simulink model "mo_hinh_dwt_wiener"  (R2026b)
settings: Solver=FixedStepDiscrete  StopTime=5.2480000000000002  FixedStep=6.2500000000000001e-05
InitFcn:
  | model = bdroot;
  | roleMatches=find_system(model,'LookUnderMasks','all','FollowLinks','off','IncludeCommented','on','Tag','WaveletDSP:source');
  | assert(numel(roleMatches)==1,'WaveletDSP:Role','Thiếu hoặc trùng định danh nội bộ: source. Không cần khôi phục tên hiển thị.');
  | source=get_param(roleMatches{1},'Handle');
  | roleMatches=find_system(model,'LookUnderMasks','all','FollowLinks','off','IncludeCommented','on','Tag','WaveletDSP:clean');
  | assert(numel(roleMatches)==1,'WaveletDSP:Role','Thiếu hoặc trùng định danh nội bộ: clean. Không cần khôi phục tên hiển thị.');
  | cleanSource=get_param(roleMatches{1},'Handle');
  | roleMatches=find_system(model,'LookUnderMasks','all','FollowLinks','off','IncludeCommented','on','Tag','WaveletDSP:sink');
  | assert(numel(roleMatches)==1,'WaveletDSP:Role','Thiếu hoặc trùng định danh nội bộ: sink. Không cần khôi phục tên hiển thị.');
  | sink=get_param(roleMatches{1},'Handle');
  | roleMatches=find_system(model,'LookUnderMasks','all','FollowLinks','off','IncludeCommented','on','Tag','WaveletDSP:filter');
  | assert(numel(roleMatches)==1,'WaveletDSP:Role','Thiếu hoặc trùng định danh nội bộ: filter. Không cần khôi phục tên hiển thị.');
  | filterBlock=get_param(roleMatches{1},'Handle');
  | roleMatches=find_system(model,'LookUnderMasks','all','FollowLinks','off','IncludeCommented','on','Tag','WaveletDSP:reference_sync');
  | assert(numel(roleMatches)==1,'WaveletDSP:Role','Thiếu hoặc trùng định danh nội bộ: reference_sync. Không cần khôi phục tên hiển thị.');
  | referenceSync=get_param(roleMatches{1},'Handle');
  | roleMatches=find_system(model,'LookUnderMasks','all','FollowLinks','off','IncludeCommented','on','Tag','WaveletDSP:noisy_sync');
  | assert(numel(roleMatches)==1,'WaveletDSP:Role','Thiếu hoặc trùng định danh nội bộ: noisy_sync. Không cần khôi phục tên hiển thị.');
  | noisySync=get_param(roleMatches{1},'Handle');
  | workspace = get_param(model,'ModelWorkspace');
  | assignin(workspace,'Export_Complete',false);
  | inputFile = get_param(source,'inputFilename');
  | inputInfo = audioinfo(inputFile);
  | assert(inputInfo.NumChannels==1,'Chỉ hỗ trợ âm thanh một kênh.');
  | useClean = strcmp(get_param(filterBlock,'Use_Clean'),'1');
  | cleanFile = get_param(cleanSource,'inputFilename');
  | if useClean && strcmp(get_param(filterBlock,'Auto_Clean'),'1')
  |     [inputFolder,inputStem] = fileparts(inputFile);
  |     recordId = regexp(inputStem,'^(speech_\d+)_','tokens','once');
  |     assert(~isempty(recordId),'Không tìm được âm thanh sạch; tắt ghép tệp tự động và chọn tệp tham chiếu trực tiếp.');
  |     cleanFile = fullfile(fileparts(fileparts(inputFolder)),'clean',[recordId{1} '.wav']);
  | end
  | frameSize = str2double(get_param(source,'SamplesPerFrame'));
  | assert(isfinite(frameSize) && frameSize>0 && mod(frameSize,128)==0,'Số mẫu mỗi khung âm thanh có nhiễu phải là bội dương của 128.');
  | if useClean
  |     cleanInfo = audioinfo(cleanFile);
  |     assert(cleanInfo.SampleRate==inputInfo.SampleRate && cleanInfo.TotalSamples==inputInfo.TotalSamples && cleanInfo.NumChannels==1,'Âm thanh sạch/noisy must match sample rate and length.');
  |     if ~strcmp(get_param(filterBlock,'Auto_Frame'),'1')
  |         assert(str2double(get_param(cleanSource,'SamplesPerFrame'))==frameSize,'Âm thanh sạch/Noisy frame sizes differ. Set them explicitly or enable Auto_Frame.');
  |     end
  | end
  | levels = [1 2 3 4 5 6 7 7];
  | powerWindow = str2double(get_param(filterBlock,'Win_Pow'));
  | smoothWindow = str2double(get_param(filterBlock,'Win_Smooth'));
  | powerLengths = max(1,round(powerWindow*inputInfo.SampleRate./2.^levels));
  | smoothLengths = max(1,round(smoothWindow*inputInfo.SampleRate./2.^levels));
  | bandDelays = floor((powerLengths-1)/2)+floor((smoothLengths-1)/2);
  | totalDelay = 29*(2^7-1)+128*ceil(max(bandDelays.*2.^levels)/128);
  | frameCount = ceil((inputInfo.TotalSamples+totalDelay)/frameSize);
  | requiredStop = (frameCount-1)*frameSize/inputInfo.SampleRate;
  | autoRun = strcmp(get_param(filterBlock,'Auto_Run'),'1');
  | if ~autoRun
  |     assert(strcmp(get_param(model,'Solver'),'FixedStepDiscrete'),'Chọn bộ giải rời rạc bước cố định hoặc bật tự tính thời gian mô phỏng.');
  |     stepValue = slResolve(get_param(model,'FixedStep'),model);
  |     stopValue = slResolve(get_param(model,'StopTime'),model);
  |     assert(isscalar(stepValue) && isfinite(stepValue) && stepValue>0 && stepValue<=1/inputInfo.SampleRate && abs((1/inputInfo.SampleRate)/stepValue-round((1/inputInfo.SampleRate)/stepValue))<1e-8,'Bước mô phỏng phải chia hết chu kỳ lấy mẫu; chỉnh bước hoặc bật tự tính thời gian.');
  |     assert(isscalar(stopValue) && isfinite(stopValue) && stopValue>=requiredStop,'Thời gian dừng quá ngắn hoặc vô hạn; đặt thời gian hữu hạn đủ dài hoặc bật tự tính thời gian.');
  | end
  | configuredOutput = get_param(sink,'outputFilename');
  | assert(~strcmp(inputFile,configuredOutput) && ~strcmp(cleanFile,configuredOutput),'Tệp đầu ra không được trùng tệp đầu vào.');
  | ... (+47 lines)
StopFcn:
  | model = bdroot;
  | workspace = get_param(model,'ModelWorkspace');
  | roleMatches=find_system(model,'LookUnderMasks','all','FollowLinks','off','IncludeCommented','on','Tag','WaveletDSP:sink');
  | assert(numel(roleMatches)==1,'WaveletDSP:Role','Thiếu hoặc trùng định danh nội bộ: sink. Không cần khôi phục tên hiển thị.');
  | sink=get_param(roleMatches{1},'Handle');
  | roleMatches=find_system(model,'LookUnderMasks','all','FollowLinks','off','IncludeCommented','on','Tag','WaveletDSP:clean');
  | assert(numel(roleMatches)==1,'WaveletDSP:Role','Thiếu hoặc trùng định danh nội bộ: clean. Không cần khôi phục tên hiển thị.');
  | cleanSource=get_param(roleMatches{1},'Handle');
  | outputFile = evalin(workspace,'Last_Output_File');
  | restoreSettings = evalin(workspace,'Run_Restore_Settings');
  | set_param(sink,'outputFilename',restoreSettings.OutputFile);
  | set_param(cleanSource,'inputFilename',restoreSettings.CleanFile,'Commented',restoreSettings.CleanCommented);
  | [outputAudio,outputRate] = audioread(outputFile);
  | delaySamples = evalin(workspace,'Total_Delay');
  | validSamples = evalin(workspace,'Valid_Samples');
  | assert(size(outputAudio,1)>=delaySamples+validSamples,'Mô phỏng dừng sớm: đầu ra chưa đủ mẫu; tệp thô được giữ lại.');
  | outputAudio = outputAudio(delaySamples+(1:validSamples),:);
  | audiowrite(outputFile,outputAudio,outputRate,'BitsPerSample',24);
  | assignin(workspace,'Export_Complete',true);
  | fprintf('Đã xuất âm thanh và giữ thiết lập. Tệp âm thanh: %s\n',outputFile);
model workspace (MAT data in the model file):
  Audio_Fs = 16000
  Export_Complete = 1
  Frame_Size = 1024
  Last_Output_File = '/home/alberttochiro/Documents/Codex/PRJ/WaveletDSP/results/denoised_output_20261108_091202_407.wav'
  Reference_Available = 1
  Run_Clean_File = '/home/alberttochiro/Documents/Codex/PRJ/WaveletDSP/data_DSP_speech/clean/speech_004.wav'
  Run_Restore_Settings : object (value not decoded)
  Total_Delay = 4579
  Valid_Samples = 79500
undefined symbols (not defined in the file or in its folder): dspblkCoreblockFVToolHelper, gcbh, Pn_1, Pn_2, Pn_3, Pn_4, Pn_5, Pn_6, Pn_7, Pn_8
libraries: dspvision x3, dspmlti4 x2, simulink x2
(part 2 of 2)

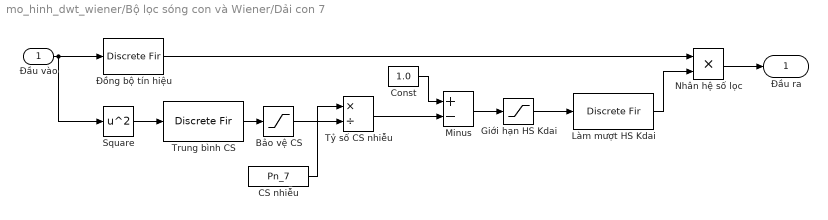
== system mo_hinh_dwt_wiener/Bộ lọc sóng con và Wiener/Dải con 7 ==
  Đầu vào : Inport
  Bảo vệ CS : Saturate  UpperLimit=inf  LowerLimit=realmin
  CS nhiễu : Constant  Value=Pn_7
  Const : Constant  Value=1.0
  Giới hạn HS Kdai : Saturate  UpperLimit=1.0  LowerLimit=Gain_Floor
  Làm mượt HS Kdai : DiscreteFir  Tag=WaveletDSP:sm_7  Coefficients=ones(1,Sample_Count)/Sample_Count  InputProcessing=Columns as channels (frame based)  mask{Sample_Count=5}
      mask prompts: Sample_Count "Số mẫu cửa sổ (tự tính từ thiết lập bộ lọc)"
      mask help: Trung bình các mẫu trong cửa sổ. Chỉnh thời gian cửa sổ tại bộ lọc; không cần nhập dãy hệ số.
      mask init:
      | validateattributes(Sample_Count,{'double'},{'scalar','integer','finite','>=',1});
  Minus : Sum  Inputs=+-
  Nhân hệ số lọc : Product
  Square : Math  Operator=square
  Trung bình CS : DiscreteFir  Tag=WaveletDSP:pow_7  Coefficients=ones(1,Sample_Count)/Sample_Count  InputProcessing=Columns as channels (frame based)  mask{Sample_Count=8}
      mask prompts: Sample_Count "Số mẫu cửa sổ (tự tính từ thiết lập bộ lọc)"
      mask help: Trung bình các mẫu trong cửa sổ. Chỉnh thời gian cửa sổ tại bộ lọc; không cần nhập dãy hệ số.
      mask init:
      | validateattributes(Sample_Count,{'double'},{'scalar','integer','finite','>=',1});
  Tỷ số CS nhiễu : Product  Inputs=*/
  Đồng bộ tín hiệu : DiscreteFir  Tag=WaveletDSP:sync_7  Coefficients=[zeros(1,Sample_Count) 1]  InputProcessing=Columns as channels (frame based)  mask{Sample_Count=5}
      mask prompts: Sample_Count "Số mẫu đồng bộ (tự tính từ cấu trúc và thiết lập bộ lọc)"
      mask help: Đồng bộ tín hiệu theo số mẫu. Giá trị được tính tự động để giữ nguyên phép lọc; không cần nhập dãy hệ số.
      mask init:
      | validateattributes(Sample_Count,{'double'},{'scalar','integer','finite','>=',0});
  Đầu ra : Outport
  wires:
  Đầu vào/1 -> Đồng bộ tín hiệu/1, Square/1
  Square/1 -> Trung bình CS/1
  Trung bình CS/1 -> Bảo vệ CS/1
  CS nhiễu/1 -> Tỷ số CS nhiễu/1
  Bảo vệ CS/1 -> Tỷ số CS nhiễu/2
  Const/1 -> Minus/1
  Tỷ số CS nhiễu/1 -> Minus/2
  Minus/1 -> Giới hạn HS Kdai/1
  Giới hạn HS Kdai/1 -> Làm mượt HS Kdai/1
  Đồng bộ tín hiệu/1 -> Nhân hệ số lọc/1
  Làm mượt HS Kdai/1 -> Nhân hệ số lọc/2
  Nhân hệ số lọc/1 -> Đầu ra/1

== system mo_hinh_dwt_wiener/Bộ lọc sóng con và Wiener/Dải con 8 ==
  Đầu vào : Inport
  Bảo vệ CS : Saturate  UpperLimit=inf  LowerLimit=realmin
  CS nhiễu : Constant  Value=Pn_8
  Const : Constant  Value=1.0
  Giới hạn HS Kdai : Saturate  UpperLimit=1.0  LowerLimit=Gain_Floor
  Làm mượt HS Kdai : DiscreteFir  Tag=WaveletDSP:sm_8  Coefficients=ones(1,Sample_Count)/Sample_Count  InputProcessing=Columns as channels (frame based)  mask{Sample_Count=5}
      mask prompts: Sample_Count "Số mẫu cửa sổ (tự tính từ thiết lập bộ lọc)"
      mask help: Trung bình các mẫu trong cửa sổ. Chỉnh thời gian cửa sổ tại bộ lọc; không cần nhập dãy hệ số.
      mask init:
      | validateattributes(Sample_Count,{'double'},{'scalar','integer','finite','>=',1});
  Minus : Sum  Inputs=+-
  Nhân hệ số lọc : Product
  Square : Math  Operator=square
  Trung bình CS : DiscreteFir  Tag=WaveletDSP:pow_8  Coefficients=ones(1,Sample_Count)/Sample_Count  InputProcessing=Columns as channels (frame based)  mask{Sample_Count=8}
      mask prompts: Sample_Count "Số mẫu cửa sổ (tự tính từ thiết lập bộ lọc)"
      mask help: Trung bình các mẫu trong cửa sổ. Chỉnh thời gian cửa sổ tại bộ lọc; không cần nhập dãy hệ số.
      mask init:
      | validateattributes(Sample_Count,{'double'},{'scalar','integer','finite','>=',1});
  Tỷ số CS nhiễu : Product  Inputs=*/
  Đồng bộ tín hiệu : DiscreteFir  Tag=WaveletDSP:sync_8  Coefficients=[zeros(1,Sample_Count) 1]  InputProcessing=Columns as channels (frame based)  mask{Sample_Count=5}
      mask prompts: Sample_Count "Số mẫu đồng bộ (tự tính từ cấu trúc và thiết lập bộ lọc)"
      mask help: Đồng bộ tín hiệu theo số mẫu. Giá trị được tính tự động để giữ nguyên phép lọc; không cần nhập dãy hệ số.
      mask init:
      | validateattributes(Sample_Count,{'double'},{'scalar','integer','finite','>=',0});
  Đầu ra : Outport
  wires:
  Đầu vào/1 -> Đồng bộ tín hiệu/1, Square/1
  Square/1 -> Trung bình CS/1
  Trung bình CS/1 -> Bảo vệ CS/1
  CS nhiễu/1 -> Tỷ số CS nhiễu/1
  Bảo vệ CS/1 -> Tỷ số CS nhiễu/2
  Const/1 -> Minus/1
  Tỷ số CS nhiễu/1 -> Minus/2
  Minus/1 -> Giới hạn HS Kdai/1
  Giới hạn HS Kdai/1 -> Làm mượt HS Kdai/1
  Đồng bộ tín hiệu/1 -> Nhân hệ số lọc/1
  Làm mượt HS Kdai/1 -> Nhân hệ số lọc/2
  Nhân hệ số lọc/1 -> Đầu ra/1

== system mo_hinh_dwt_wiener/Bộ đo chỉ số/Mẫu hợp lệ ==
  Bảo vệ số mẫu : Saturate  UpperLimit=inf  LowerLimit=realmin
  Chỉ số mẫu : Bias  Bias=(0:Frame_Size-1)'  SaturateOnIntegerOverflow=off
  Mẫu được tính : Logic  AllPortsSameDT=off  OutDataTypeStr=boolean
  Sau điểm bắt đầu : simulink/Logic and Bit Operations/Compare To Constant  relop=>=  const=Total_Delay  OutDataTypeStr=boolean
  Thời gian khung : DigitalClock  SampleTime=Frame_Size/Audio_Fs
  Trước điểm kết thúc : simulink/Logic and Bit Operations/Compare To Constant  relop=<  const=Total_Delay+Valid_Samples  OutDataTypeStr=boolean
  Tích lũy số mẫu : DiscreteFilter  Numerator=1  Denominator=[1 -1]
  Tổng theo khung số mẫu : Gain  Gain=ones(1,Frame_Size)  Multiplication=Matrix(K*u)
  Vị trí đầu khung : Gain  Gain=Audio_Fs
  Đổi kiểu mẫu hợp lệ : DataTypeConversion  OutDataTypeStr=double  SaturateOnIntegerOverflow=off  RndMeth=Floor
  Output 1 : Outport
  Output 2 : Outport  Port=2
  Output 3 : Outport  Port=3
  wires:
  Trước điểm kết thúc/1 -> Mẫu được tính/2
  Đổi kiểu mẫu hợp lệ/1 -> Output 1/1, Tổng theo khung số mẫu/1
  Tích lũy số mẫu/1 -> Output 3/1, Bảo vệ số mẫu/1
  Tổng theo khung số mẫu/1 -> Tích lũy số mẫu/1
  Mẫu được tính/1 -> Đổi kiểu mẫu hợp lệ/1
  Vị trí đầu khung/1 -> Chỉ số mẫu/1
  Chỉ số mẫu/1 -> Sau điểm bắt đầu/1, Trước điểm kết thúc/1
  Thời gian khung/1 -> Vị trí đầu khung/1
  Sau điểm bắt đầu/1 -> Mẫu được tính/1
  Bảo vệ số mẫu/1 -> Output 2/1

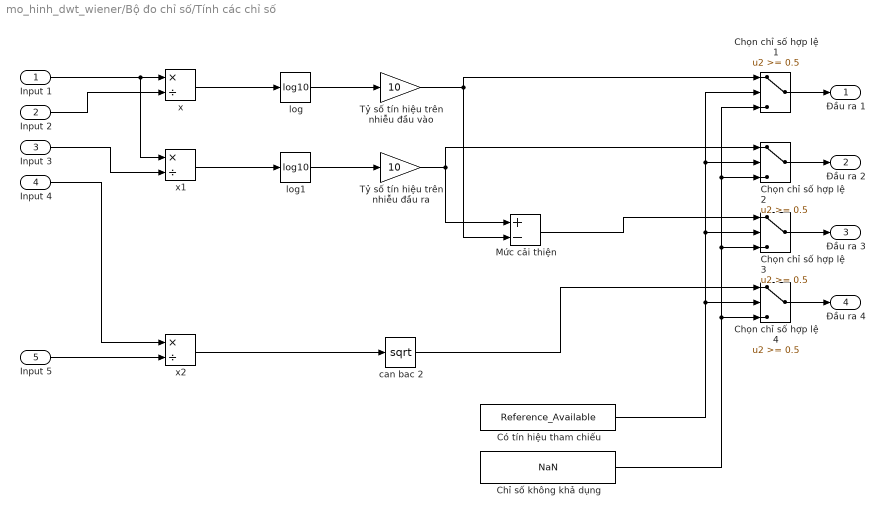
== system mo_hinh_dwt_wiener/Bộ đo chỉ số/Tính các chỉ số ==
  Input 1 : Inport
  Input 2 : Inport  Port=2
  Input 3 : Inport  Port=3
  Input 4 : Inport  Port=4
  Input 5 : Inport  Port=5
  Chỉ số không khả dụng : Constant  Value=NaN
  Chọn chỉ số hợp lệ {1..4} (4 alike) : Switch  Threshold=0.5  SaturateOnIntegerOverflow=off  InputSameDT=off
  Có tín hiệu tham chiếu : Constant  Value=Reference_Available
  Mức cải thiện : Sum  Inputs=+-
  Tỷ số tín hiệu trên nhiễu đầu ra : Gain  Gain=10
  Tỷ số tín hiệu trên nhiễu đầu vào : Gain  Gain=10
  can bac 2 : Math  Operator=sqrt
  log : Math  Operator=log10
  log1 : Math  Operator=log10
  x : Product  Inputs=*/
  x1 : Product  Inputs=*/
  x2 : Product  Inputs=*/
  Đầu ra 1 : Outport
  Đầu ra 2 : Outport  Port=2
  Đầu ra 3 : Outport  Port=3
  Đầu ra 4 : Outport  Port=4
  wires:
  x1/1 -> log1/1
  Input 3/1 -> x1/2
  Chọn chỉ số hợp lệ 4/1 -> Đầu ra 4/1
  Có tín hiệu tham chiếu/1 -> Chọn chỉ số hợp lệ 1/2, Chọn chỉ số hợp lệ 2/2, Chọn chỉ số hợp lệ 3/2, Chọn chỉ số hợp lệ 4/2
  log/1 -> Tỷ số tín hiệu trên nhiễu đầu vào/1
  Input 5/1 -> x2/2
  x/1 -> log/1
  Mức cải thiện/1 -> Chọn chỉ số hợp lệ 3/1
  Chọn chỉ số hợp lệ 2/1 -> Đầu ra 2/1
  Chọn chỉ số hợp lệ 1/1 -> Đầu ra 1/1
  Input 4/1 -> x2/1
  Chọn chỉ số hợp lệ 3/1 -> Đầu ra 3/1
  can bac 2/1 -> Chọn chỉ số hợp lệ 4/1
  Input 1/1 -> x1/1, x/1
  log1/1 -> Tỷ số tín hiệu trên nhiễu đầu ra/1
  Tỷ số tín hiệu trên nhiễu đầu ra/1 -> Mức cải thiện/1, Chọn chỉ số hợp lệ 2/1
  x2/1 -> can bac 2/1
  Tỷ số tín hiệu trên nhiễu đầu vào/1 -> Chọn chỉ số hợp lệ 1/1, Mức cải thiện/2
  Input 2/1 -> x/2
  Chỉ số không khả dụng/1 -> Chọn chỉ số hợp lệ 3/3, Chọn chỉ số hợp lệ 1/3, Chọn chỉ số hợp lệ 2/3, Chọn chỉ số hợp lệ 4/3

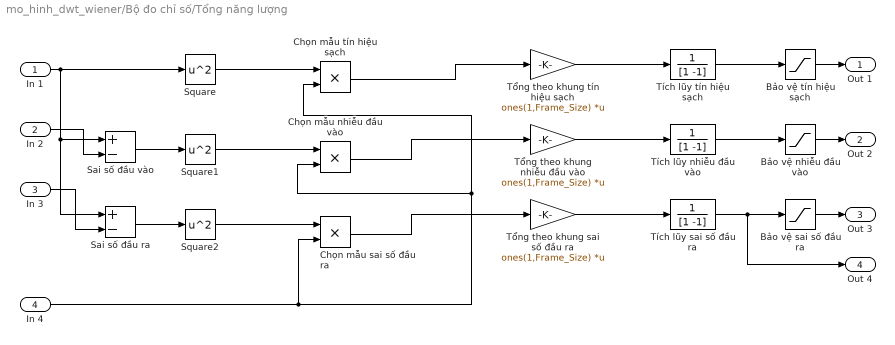
== system mo_hinh_dwt_wiener/Bộ đo chỉ số/Tổng năng lượng ==
  In 1 : Inport
  In 2 : Inport  Port=2
  In 3 : Inport  Port=3
  In 4 : Inport  Port=4
  Bảo vệ nhiễu đầu vào : Saturate  UpperLimit=inf  LowerLimit=realmin
  Bảo vệ sai số đầu ra : Saturate  UpperLimit=inf  LowerLimit=realmin
  Bảo vệ tín hiệu sạch : Saturate  UpperLimit=inf  LowerLimit=realmin
  Chọn mẫu nhiễu đầu vào : Product
  Chọn mẫu sai số đầu ra : Product
  Chọn mẫu tín hiệu sạch : Product
  Sai số đầu ra : Sum  Inputs=+-
  Sai số đầu vào : Sum  Inputs=+-
  Square : Math  Operator=square
  Square1 : Math  Operator=square
  Square2 : Math  Operator=square
  Tích lũy nhiễu đầu vào : DiscreteFilter  Numerator=1  Denominator=[1 -1]
  Tích lũy sai số đầu ra : DiscreteFilter  Numerator=1  Denominator=[1 -1]
  Tích lũy tín hiệu sạch : DiscreteFilter  Numerator=1  Denominator=[1 -1]
  Tổng theo khung nhiễu đầu vào : Gain  Gain=ones(1,Frame_Size)  Multiplication=Matrix(K*u)
  Tổng theo khung sai số đầu ra : Gain  Gain=ones(1,Frame_Size)  Multiplication=Matrix(K*u)
  Tổng theo khung tín hiệu sạch : Gain  Gain=ones(1,Frame_Size)  Multiplication=Matrix(K*u)
  Out 1 : Outport
  Out 2 : Outport  Port=2
  Out 3 : Outport  Port=3
  Out 4 : Outport  Port=4
  wires:
  Sai số đầu ra/1 -> Square2/1
  Tích lũy nhiễu đầu vào/1 -> Bảo vệ nhiễu đầu vào/1
  Chọn mẫu tín hiệu sạch/1 -> Tổng theo khung tín hiệu sạch/1
  Tích lũy tín hiệu sạch/1 -> Bảo vệ tín hiệu sạch/1
  Sai số đầu vào/1 -> Square1/1
  In 3/1 -> Sai số đầu ra/2
  In 1/1 -> Sai số đầu vào/1, Sai số đầu ra/1, Square/1
  In 4/1 -> Chọn mẫu tín hiệu sạch/2, Chọn mẫu nhiễu đầu vào/2, Chọn mẫu sai số đầu ra/2
  Bảo vệ sai số đầu ra/1 -> Out 3/1
  Square/1 -> Chọn mẫu tín hiệu sạch/1
  Tổng theo khung nhiễu đầu vào/1 -> Tích lũy nhiễu đầu vào/1
  Chọn mẫu nhiễu đầu vào/1 -> Tổng theo khung nhiễu đầu vào/1
  Square1/1 -> Chọn mẫu nhiễu đầu vào/1
  In 2/1 -> Sai số đầu vào/2
  Tổng theo khung tín hiệu sạch/1 -> Tích lũy tín hiệu sạch/1
  Chọn mẫu sai số đầu ra/1 -> Tổng theo khung sai số đầu ra/1
  Bảo vệ nhiễu đầu vào/1 -> Out 2/1
  Tổng theo khung sai số đầu ra/1 -> Tích lũy sai số đầu ra/1
  Square2/1 -> Chọn mẫu sai số đầu ra/1
  Bảo vệ tín hiệu sạch/1 -> Out 1/1
  Tích lũy sai số đầu ra/1 -> Bảo vệ sai số đầu ra/1, Out 4/1
